simulink model "CabinGuard_MATLAB_simulation"  (R2024a)
settings: Solver=ode4  StartTime=0.0  StopTime=45  FixedStep=0.01  RelTol=1e-3
undefined symbols (not defined in the file or in its folder): ca_a_comf, ca_a_lo, ca_absvel, ca_clear, ca_d0, ca_det, ca_edge, ca_ego_id, ca_go_phase, ca_hw, ca_jdn, ca_jup, ca_kfeas, ca_lka_in, ca_lka_out, ca_lw0, ca_min_shift, ca_plant, ca_psi0, ca_pv, ca_sys, ca_t_act, ca_v0, ca_vlat, ca_wn, ca_X0, ca_Y0, driving, matlabshared
libraries: simulink x102, drivingscenarioandsensors x5, autolibshared x2, mpcadaslib x1, slpidlib x1
(part 1 of 4)
settings Model: SimulationMode=accelerator  Creator=anonymous  LastModifiedBy=anonymous
settings DebuggingCC: BusObjectLabelMismatch=none

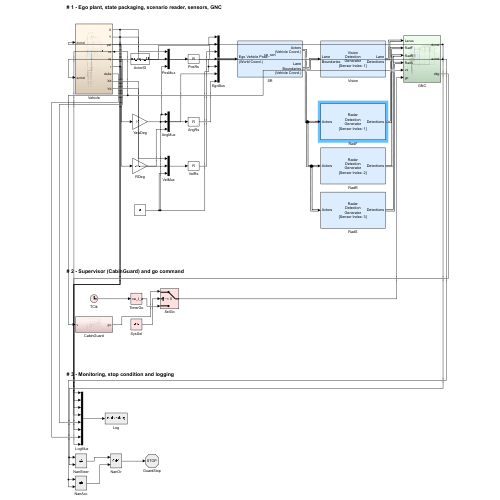
[thumbnail: Simulink's stored preview of the top-level diagram]
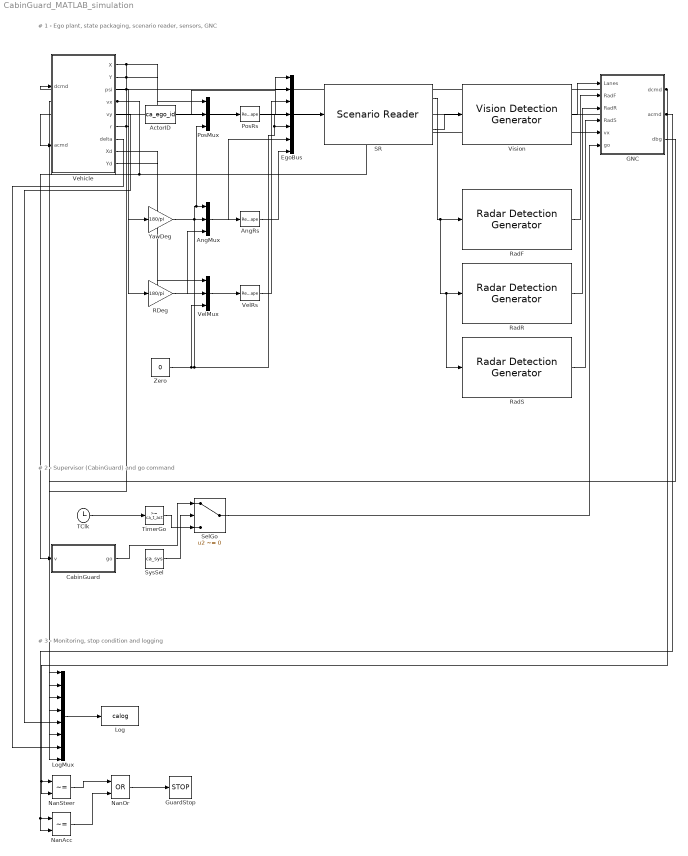
== system CabinGuard_MATLAB_simulation ==
  note: # 1 - Ego plant, state packaging, scenario reader, sensors, GNC
  note: # 2 - Supervisor (CabinGuard) and go command
  note: # 3 - Monitoring, stop condition and logging
  ActorID : Constant  Value=ca_ego_id
  AngMux : Mux  Inputs=3
  AngRs : Reshape  OutputDimensionality=Customize  OutputDimensions=[1 3]
  CabinGuard : Subsystem
  EgoBus : BusCreator  Inputs=7  OutDataTypeStr=Bus: cgEgoIn
  GNC : Subsystem
  GuardStop : Stop
  Log : ToWorkspace  VariableName=calog  SampleTime=0.02
  LogMux : Mux  Inputs=8
  NanAcc : RelationalOperator  Operator=~=  OutDataTypeStr=boolean  RndMeth=Simplest  InputSameDT=off
  NanOr : Logic  Operator=OR  AllPortsSameDT=off  OutDataTypeStr=boolean
  NanSteer : RelationalOperator  Operator=~=  OutDataTypeStr=boolean  RndMeth=Simplest  InputSameDT=off
  PosMux : Mux  Inputs=3
  PosRs : Reshape  OutputDimensionality=Customize  OutputDimensions=[1 3]
  RDeg : Gain  Gain=180/pi
  RadF : drivingscenarioandsensors/Radar Detection Generator  SensorIndex=1  UpdateInterval=0.1  SensorLocation=[3.7 0]  Height=0.2  Yaw=0  Pitch=0  Roll=0  BusNameSource=Auto  BusName=BusRadarDetectionGenerator  MaxNumDetectionsSource=Property  MaxNumDetections=6  DetectionCoordinates=Ego Cartesian  SimulateUsing=Interpreted execution  AzimuthResolution=4  ElevationResolution=10  RangeResolution=2.5  RangeRateResolution=0.5  AzimuthBiasFraction=0.1  ElevationBiasFraction=0.1  RangeBiasFraction=0.05  RangeRateBiasFraction=0.05  FieldOfView=[100 10]  MaxRange=150  RangeRateLimits=[ -100, 100 ]  DetectionProbability=0.9  FalseAlarmRate=1e-6  ReferenceRange=100  ReferenceRCS=0  HasElevation=off  HasRangeRate=on  HasNoise=on  HasFalseAlarms=off  HasOcclusion=on  InitialSeedSource=Repeatable  InitialSeed=0  UsedSeed=matlabshared.tracking.internal.SimulinkUtilities.seedManager(gcb)  ActorProfilesSource=Parameters  ActorProfilesParameters=driving.internal.ActorProfilesRadarParameters  ActorProfilesExpression=struct( 'ClassID', 0, 'Length', 4.7, 'Width', 1.8, 'Height', 1.4, 'OriginOffset', [ -1.35, 0, 0 ], 'RCSPattern', [ 10, 10; 10, 10 ], 'RCSAzimuthAngles', [ -180, 180 ], 'RCSElevationAngles', [ -90, 90 ] )
  RadR : drivingscenarioandsensors/Radar Detection Generator  SensorIndex=2  UpdateInterval=0.1  SensorLocation=[-1 0]  Height=0.2  Yaw=180  Pitch=0  Roll=0  BusNameSource=Auto  BusName=BusRadarDetectionGenerator  MaxNumDetectionsSource=Property  MaxNumDetections=6  DetectionCoordinates=Ego Cartesian  SimulateUsing=Interpreted execution  AzimuthResolution=4  ElevationResolution=10  RangeResolution=2.5  RangeRateResolution=0.5  AzimuthBiasFraction=0.1  ElevationBiasFraction=0.1  RangeBiasFraction=0.05  RangeRateBiasFraction=0.05  FieldOfView=[60 10]  MaxRange=120  RangeRateLimits=[ -100, 100 ]  DetectionProbability=0.9  FalseAlarmRate=1e-6  ReferenceRange=100  ReferenceRCS=0  HasElevation=off  HasRangeRate=on  HasNoise=on  HasFalseAlarms=off  HasOcclusion=on  InitialSeedSource=Repeatable  InitialSeed=0  UsedSeed=matlabshared.tracking.internal.SimulinkUtilities.seedManager(gcb)  ActorProfilesSource=Parameters  ActorProfilesParameters=driving.internal.ActorProfilesRadarParameters  ActorProfilesExpression=struct( 'ClassID', 0, 'Length', 4.7, 'Width', 1.8, 'Height', 1.4, 'OriginOffset', [ -1.35, 0, 0 ], 'RCSPattern', [ 10, 10; 10, 10 ], 'RCSAzimuthAngles', [ -180, 180 ], 'RCSElevationAngles', [ -90, 90 ] )
  RadS : drivingscenarioandsensors/Radar Detection Generator  SensorIndex=3  UpdateInterval=0.1  SensorLocation=[2.0 -0.9]  Height=0.2  Yaw=-90  Pitch=0  Roll=0  BusNameSource=Auto  BusName=BusRadarDetectionGenerator  MaxNumDetectionsSource=Property  MaxNumDetections=6  DetectionCoordinates=Ego Cartesian  SimulateUsing=Interpreted execution  AzimuthResolution=4  ElevationResolution=10  RangeResolution=2.5  RangeRateResolution=0.5  AzimuthBiasFraction=0.1  ElevationBiasFraction=0.1  RangeBiasFraction=0.05  RangeRateBiasFraction=0.05  FieldOfView=[150 10]  MaxRange=30  RangeRateLimits=[ -100, 100 ]  DetectionProbability=0.9  FalseAlarmRate=1e-6  ReferenceRange=100  ReferenceRCS=0  HasElevation=off  HasRangeRate=on  HasNoise=on  HasFalseAlarms=off  HasOcclusion=on  InitialSeedSource=Repeatable  InitialSeed=0  UsedSeed=matlabshared.tracking.internal.SimulinkUtilities.seedManager(gcb)  ActorProfilesSource=Parameters  ActorProfilesParameters=driving.internal.ActorProfilesRadarParameters  ActorProfilesExpression=struct( 'ClassID', 0, 'Length', 4.7, 'Width', 1.8, 'Height', 1.4, 'OriginOffset', [ -1.35, 0, 0 ], 'RCSPattern', [ 10, 10; 10, 10 ], 'RCSAzimuthAngles', [ -180, 180 ], 'RCSElevationAngles', [ -90, 90 ] )
  SR : drivingscenarioandsensors/Scenario Reader  ScenarioSource=From workspace  ScenarioFileName=EgoVehicleGoesStraight.mat  ScenarioVariableName=ca_scn  OutputCoordinateSystem=Vehicle coordinates  EgoVehicleSource=Input port  EgoVehicleActorID=1  OrientVehiclesOnRoad=off  OutputEgoVehiclePose=off  OutputEgoVehicleState=off  SampleTime=0.1  LaneBoundaryOutput=Ego vehicle lane boundaries  LaneBoundaryDistance=0:1:30  LaneBoundaryLocation=Center of lane markings  BusNameSource=Auto  BusName=BusActors  BusNumActorsSource=Scenario  BusNumActors=100  BusName2Source=Auto  BusName2=BusLaneBoundaries  BusNumLaneBoundariesSource=Scenario  BusNumLaneBoundaries=10  BusName3Source=Auto  BusName3=BusEgoActor  BusName4Source=Auto  BusName4=BusEgoState  ShowCoordinateLabels=on  SimulateUsing=Interpreted execution
  SelGo : Switch  Criteria=u2 ~= 0  SaturateOnIntegerOverflow=off  InputSameDT=off
  SysSel : Constant  Value=ca_sys
  TClk : Clock
  TimerGo : simulink/Logic and Bit Operations/Compare To Constant  relop=>=  const=ca_t_act  OutDataTypeStr=boolean
  Vehicle : Subsystem
  VelMux : Mux  Inputs=3
  VelRs : Reshape  OutputDimensionality=Customize  OutputDimensions=[1 3]
  Vision : drivingscenarioandsensors/Vision Detection Generator  SensorIndex=1  DetectorOutput=Lanes only  UpdateInterval=0.1  LaneUpdateInterval=0.1  SensorLocation=[ 1.9, 0 ]  Height=1.1  Yaw=0  Pitch=1  Roll=0  BusNameSource=Auto  BusName=BusObjectDetections  BusName2Source=Auto  BusName2=BusLaneDetections  MaxNumDetectionsSource=Property  MaxNumDetections=50  MaxNumLanesSource=Property  MaxNumLanes=30  DetectionCoordinates=Ego Cartesian  SimulateUsing=Interpreted execution  MaxRange=150  BoundingBoxAccuracy=5  ProcessNoiseIntensity=5  MaxSpeed=100  MaxAllowedOcclusion=0.5  MinObjectImageSize=[ 15, 15 ]  DetectionProbability=0.9  FalsePositivesPerImage=0.1  MinLaneImageSize=[ 20, 3 ]  LaneBoundaryAccuracy=3  HasNoise=on  InitialSeedSource=Repeatable  InitialSeed=0  UsedSeed=driving.internal.SimulinkUtilities.seedManager(gcb)  ActorProfilesSource=From Scenario Reader block  ActorProfilesParameters=driving.internal.ActorProfilesParameters  ActorProfilesExpression=struct( 'ClassID', 0, 'Length', 4.7, 'Width', 1.8, 'Height', 1.4, 'OriginOffset', [ -1.35, 0, 0 ] )  Intrinsics=driving.internal.cameraIntrinsics
  YawDeg : Gain  Gain=180/pi
  Zero : Constant  Value=0
  wires:
  AngRs/1 -> EgoBus/7
  Vehicle/1(X) -> PosMux/1, LogMux/1
  YawDeg/1 -> EgoBus/6
  TimerGo/1 -> SelGo/3
  Vehicle/2(Y) -> PosMux/2, LogMux/2
  Vehicle/4(vx) -> GNC/5(vx), CabinGuard/1(v), LogMux/4
  Vehicle/3(psi) -> YawDeg/1, LogMux/3
  Vehicle/5(vy) -> LogMux/5
  Vehicle/7(delta) -> LogMux/7
  Vehicle/6(r) -> LogMux/6, RDeg/1
  Vehicle/8(Xd) -> VelMux/1
  Vehicle/9(Yd) -> VelMux/2
  TClk/1 -> TimerGo/1
  SelGo/1 -> GNC/6(go)
  Zero/1 -> EgoBus/4, EgoBus/5, PosMux/3, AngMux/1, AngMux/2, VelMux/3
  PosRs/1 -> EgoBus/2
  RDeg/1 -> AngMux/3
  CabinGuard/1(go) -> SelGo/1
  SysSel/1 -> SelGo/2
  VelRs/1 -> EgoBus/3
  PosMux/1 -> PosRs/1
  AngMux/1 -> AngRs/1
  VelMux/1 -> VelRs/1
  ActorID/1 -> EgoBus/1
  Vision/1 -> GNC/1(Lanes)
  EgoBus/1 -> SR/1
  SR/2 -> Vision/1
  SR/1 -> RadR/1, RadS/1, RadF/1
  RadF/1 -> GNC/2(RadF)
  NanAcc/1 -> NanOr/2
  NanSteer/1 -> NanOr/1
  RadR/1 -> GNC/3(RadR)
  RadS/1 -> GNC/4(RadS)
  GNC/1(dcmd) -> NanSteer/2, NanSteer/1, Vehicle/1(dcmd)
  GNC/2(acmd) -> NanAcc/1, NanAcc/2, Vehicle/2(acmd)
  GNC/3(dbg) -> LogMux/8
  LogMux/1 -> Log/1
  NanOr/1 -> GuardStop/1

== system CabinGuard_MATLAB_simulation/CabinGuard ==
  v : Inport
  Clk : DigitalClock  SampleTime=0.01
  DP : Constant  Value=ca_det(:)
  Det : MATLAB Function  TreatAsAtomicUnit=on
  Drv : MATLAB Function  TreatAsAtomicUnit=on
  Flt : MATLAB Function  TreatAsAtomicUnit=on
  GoCmp : simulink/Logic and Bit Operations/Compare To Constant  relop=>=  const=ca_go_phase  OutDataTypeStr=boolean
  GoD : DataTypeConversion  OutDataTypeStr=double  SaturateOnIntegerOverflow=off  RndMeth=Floor
  Gw : MATLAB Function  TreatAsAtomicUnit=on
  Host : MATLAB Function  TreatAsAtomicUnit=on
  LogMux : Mux  Inputs=18
  PV : Constant  Value=ca_pv(:)
  SysLog : ToWorkspace  VariableName=syslog  SampleTime=0.02
  T{1..6} (6 alike) : Terminator
  Tel : MATLAB Function  TreatAsAtomicUnit=on
  Vz : ZeroOrderHold  SampleTime=0.01
  Zero : Constant  Value=0
  go : Outport
  wires:
  v/1 -> Vz/1
  GoD/1 -> LogMux/4
  Clk/1 -> Gw/1(t), Tel/1(t), Host/1(t), Drv/1(t), Flt/1(t), Det/1(t), LogMux/1
  Tel/1(delivered) -> LogMux/7
  DP/1 -> Det/3(dp)
  Det/1(lam) -> Flt/2(lam)
  Drv/5(clonic) -> Host/6(clonic)
  Zero/1 -> Drv/3(psi), Drv/2(y)
  Flt/4(cell_up) -> Tel/5(cell_up)
  PV/1 -> Drv/5(pv), Flt/3(pv), Host/9(pv), Det/2(pv), Gw/5(pv)
  Gw/6(alive_lost) -> LogMux/10
  Vz/1 -> Drv/4(v), Host/8(v), Gw/4(v)
  Flt/1(lam_f) -> Host/2(lam)
  Flt/2(avail) -> Host/3(avail)
  Flt/3(att) -> Gw/3(att)
  Flt/5(sms_up) -> Tel/6(sms_up)
  Drv/1(steer) -> T1/1
  Drv/2(a_drv) -> T2/1
  Host/2(F) -> T3/1
  Drv/3(tau) -> LogMux/16, Host/4(tau)
  Drv/4(brake_pedal) -> LogMux/17, Host/7(brake_pedal)
  Drv/6(grip) -> LogMux/18, Host/5(grip)
  Gw/1(a_mrm) -> LogMux/15
  Host/1(hf) -> Gw/2(hf)
  Host/3(alert) -> LogMux/5
  Host/4(dmode) -> LogMux/11
  Host/5(Pmax) -> LogMux/12, Tel/4(Pmax)
  Host/6(cls) -> LogMux/13, Tel/3(cls)
  Host/7(ecall) -> LogMux/6, Tel/2(ecall)
  Host/8(warn) -> LogMux/14
  Host/9(state) -> LogMux/2
  Gw/2(gwp_out) -> LogMux/3, GoCmp/1
  Gw/3(lk_on) -> T4/1
  Gw/4(y_ref) -> T5/1
  Gw/5(park_out) -> T6/1
  Gw/7(reject) -> LogMux/8
  Gw/8(nrej_out) -> LogMux/9
  GoCmp/1 -> go/1, GoD/1
  LogMux/1 -> SysLog/1

== system CabinGuard_MATLAB_simulation/GNC ==
  note: # GNC pipeline: Navigation -> Perception -> Decision -> Guidance -> Control
  note: # Debug bus
  Lanes : Inport
  RadF : Inport  Port=2
  RadR : Inport  Port=3
  RadS : Inport  Port=4
  vx : Inport  Port=5
  go : Inport  Port=6
  Control : Subsystem
  DbgMux : Mux  Inputs=13
  Decision : Subsystem
  Guidance : Subsystem
  Navigation : Subsystem
  OccD : DataTypeConversion  OutDataTypeStr=double  SaturateOnIntegerOverflow=off  RndMeth=Floor
  Perception : Subsystem
  dcmd : Outport
  acmd : Outport  Port=2
  dbg : Outport  Port=3
  wires:
  Lanes/1 -> Navigation/1(Lanes)
  Guidance/4(aref) -> DbgMux/5, Control/8(aref)
  RadR/1 -> Perception/2(RR)
  vx/1 -> Navigation/2(vx)
  Navigation/5(d) -> Control/1(d), DbgMux/2
  Navigation/1(e1) -> DbgMux/1
  Navigation/2(e2) -> Control/2(e2)
  Navigation/4(vmeas) -> Control/4(vmeas), Decision/3(vmeas), Perception/5(vmeas)
  Navigation/3(kappa) -> Control/3(kappa), Perception/4(kappa)
  RadF/1 -> Perception/1(RF)
  RadS/1 -> Perception/3(RS)
  go/1 -> Guidance/3(go), Decision/4(go)
  Guidance/1(yref) -> DbgMux/3, Control/5(yref)
  Perception/1(areq) -> DbgMux/8, Decision/1(areq)
  Guidance/2(ydot) -> Control/6(ydot)
  Perception/2(occ) -> OccD/1, Decision/2(occ)
  Guidance/8(lo) -> Control/11(lo)
  Guidance/6(actd) -> DbgMux/6
  Decision/1(ulat) -> Guidance/2(ulat)
  Decision/2(adem) -> DbgMux/7, Guidance/1(adem)
  Control/1(dcmd) -> DbgMux/13, dcmd/1
  Decision/4(yshT) -> DbgMux/11
  Decision/5(commit) -> DbgMux/10
  Control/2(acmd) -> DbgMux/12, acmd/1
  Guidance/3(vref) -> DbgMux/4, Control/7(vref)
  Guidance/5(act) -> Control/9(act)
  Guidance/7(up) -> Control/10(up)
  DbgMux/1 -> dbg/1
  OccD/1 -> DbgMux/9
